simulink model "ATOM_parking_chain"  (R2026a)
settings: Solver=ode4  StopTime=100  FixedStep=0.01
StopFcn:
  | % Put every new figure in the same MATLAB Figures window as a docked tab.
  | set(groot, 'defaultFigureWindowStyle', 'docked');
  | 
  | if exist('costmap_active', 'var') && ...
  |         exist('vehicle', 'var') && ...
  |         exist('parking_path', 'var') && ...
  |         ~isempty(parking_path)
  | 
  |     plotPlan(costmap_active, vehicle, parking_path);
  | 
  | else
  | 
  |     warning('No valid parking path is available for plotting.');
  | 
  | end
  | 
  | PlotControllerReferences( ...
  |     out.controller_reference_log);
  | 
  | PlotControllerTracking( ...
  |     out.controller_tracking_log);
undefined symbols (not defined in the file): lateral, longitudinal, stanley, vehicle
(part 11 of 11)

== matlab function ATOM_parking_chain/steeringRatetoAngle2/steeringRateToAngle ==
  settings: updateMethod=DISCRETE  sampleTime=0.04
  data: df_rate_cmd input; df_angle_cmd output; dr_rate_cmd input; df_measured input; dr_measured input; sample_time input; steer_rate_limit input; steer_angle_limit input; dr_angle_cmd output
function [df_angle_cmd, dr_angle_cmd] = steeringRateToAngle( ...
    df_rate_cmd, dr_rate_cmd, df_measured, dr_measured, ...
    sample_time, steer_rate_limit, steer_angle_limit)

persistent df_command_state dr_command_state

% Initialize the commanded angles from the measured wheel angles.
if isempty(df_command_state)
    df_command_state = max( ...
        -steer_angle_limit, ...
        min(steer_angle_limit,df_measured));

    dr_command_state = max( ...
        -steer_angle_limit, ...
        min(steer_angle_limit,dr_measured));
end

% Apply hard steering-rate limits.
front_rate = max( ...
    -steer_rate_limit, ...
    min(steer_rate_limit,df_rate_cmd));

rear_rate = max( ...
    -steer_rate_limit, ...
    min(steer_rate_limit,dr_rate_cmd));

% Integrate rates into desired steering angles.
df_command_state = df_command_state + sample_time*front_rate;
dr_command_state = dr_command_state + sample_time*rear_rate;

% Apply hard steering-angle limits.
df_command_state = max( ...
    -steer_angle_limit, ...
    min(steer_angle_limit,df_command_state));

dr_command_state = max( ...
    -steer_angle_limit, ...
    min(steer_angle_limit,dr_command_state));

df_angle_cmd = df_command_state;
dr_angle_cmd = dr_command_state;

end

== matlab function ATOM_parking_chain/time_parameterization2/Time parameterization ==
  data: trajectory_in input Bus: TrajectoryDataBus size=1; reference_out output Bus: ParkingReferenceBus size=1; steer_rate_limit input
function reference_out = timeParameterization( ...
    trajectory_in,steer_rate_limit)
%#codegen
%
% Convert the 100-point spatial parking trajectory into a nominal
% time-parameterized reference trajectory.

N = 100;

%% Extract the smoothed trajectory

x_ref = trajectory_in.pose.position.x;
y_ref = trajectory_in.pose.position.y;

qz = trajectory_in.pose.orientation.qz;
qw = trajectory_in.pose.orientation.qw;

v_ref = trajectory_in.longitudinal_velocity_mps;
a_ref = trajectory_in.acceleration_mps2;

df_plan = trajectory_in.front_wheel_angle_rad;
dr_plan = trajectory_in.rear_wheel_angle_rad;

rear_angle = trajectory_in.rear_wheel_angle_rad;

%% Convert quaternion to continuous body-heading reference

psi_ref = zeros(N,1);

psi_ref(1) = 2.0*atan2(qz(1),qw(1));

for k = 2:N

    raw_heading = 2.0*atan2(qz(k),qw(k));

    heading_change = raw_heading-psi_ref(k-1);

    psi_ref(k) = ...
        raw_heading-2.0*pi*round(heading_change/(2.0*pi));
end

%% Calculate distance and nominal time

s_ref = zeros(N,1);
t_ref = zeros(N,1);

for k = 1:N-1

    dx = x_ref(k+1)-x_ref(k);
    dy = y_ref(k+1)-y_ref(k);

    ds = hypot(dx,dy);

    s_ref(k+1) = s_ref(k)+ds;

    % Convert signed body-longitudinal velocity to positive rear-axle
    % path speed.
    path_speed_current = ...
        abs(v_ref(k))/max(cos(rear_angle(k)),0.1);

    path_speed_next = ...
        abs(v_ref(k+1))/max(cos(rear_angle(k+1)),0.1);

    speed_sum = path_speed_current+path_speed_next;

    if ds <= 1e-9

        dt = 0.0;

    elseif speed_sum > 1e-6

        % ds = 0.5*(v_current+v_next)*dt
        dt = 2.0*ds/speed_sum;

    else

        % Protect against an interval whose two endpoint speeds are zero.
        fallback_path_speed = 0.05;

        dt = ds/fallback_path_speed;
    end

    t_ref(k+1) = t_ref(k)+dt;
end
N = numel(t_ref);

df_nom = zeros(size(df_plan));
dr_nom = zeros(size(dr_plan));

% Start from the planner's first steering configuration.
df_nom(1) = df_plan(1);
dr_nom(1) = dr_plan(1);

for i = 2:N

    dt = max(t_ref(i)-t_ref(i-1),0.0);
    maximum_change = steer_rate_limit*dt;

    front_difference = df_plan(i)-df_nom(i-1);
    rear_difference  = dr_plan(i)-dr_nom(i-1);

    front_change = max( ...
        -maximum_change, ...
        min(maximum_change,front_difference));

    rear_change = max( ...
        -maximum_change, ...
        min(maximum_change,rear_difference));

    df_nom(i) = df_nom(i-1)+front_change;
    dr_nom(i) = dr_nom(i-1)+rear_change;

end

reference_out.t_ref   = t_ref;
reference_out.s_ref   = s_ref;
reference_out.x_ref   = x_ref;
reference_out.y_ref   = y_ref;
reference_out.psi_ref = psi_ref;
reference_out.v_ref   = v_ref;
reference_out.a_ref   = a_ref;
% Temporary pass-through. The next step will make these rate-feasible.
reference_out.df_nom = df_nom;
reference_out.dr_nom = dr_nom;
end

== matlab function ATOM_parking_chain/Parking Scenario1/Costmap generation: corridor occupancy grid/MATLAB Function ==
  data: veh input; costmap output Bus: OccupancyGridBus; start_pose output; goal_pose output
function [costmap, start_pose, goal_pose] = costmapNarrowCorridor(veh) %#ok<INUSD>
%COSTMAPNARROWCORRIDOR  8 m wide corridor.
%
% The planner turns in 5.47 m and the car is 2.66 m wide with its margin,
% so this corridor allows driving through but not turning around.
% Default task is a straight transit, which succeeds.
%
% To make it the limit case, change goal_pose heading to -pi/2 - a U-turn.
% That is expected to FAIL with a 5.47 m radius, and it is exactly the
% case a tighter turning circle would change.

persistent occ

res = 0.3;   W = 234;   H = 234;
origin_x = -(W/2)*res;
origin_y = -(H/2)*res;

if isempty(occ)
    [IX, IY] = meshgrid(0:W-1, 0:H-1);
    X = origin_x + IX*res;
    Y = origin_y + IY*res;

    lot_x = [ -4   4   4  -4];
    lot_y = [-12 -12  12  12];
    occ = ones(H,W);
    occ(inpolygon(X, Y, lot_x, lot_y)) = 0;
end

start_pose = [0, -8, pi/2];
goal_pose  = [0,  6, pi/2];

costmap.info.resolution           = res;
costmap.info.width                = uint32(W);
costmap.info.height               = uint32(H);
costmap.info.origin.position.x    = origin_x;
costmap.info.origin.position.y    = origin_y;
costmap.info.origin.position.z    = 0;
costmap.info.origin.orientation.x = 0;
costmap.info.origin.orientation.y = 0;
costmap.info.origin.orientation.z = 0;
costmap.info.origin.orientation.w = 1;
costmap.data                      = int8(occ*100);
end
